simulink model "L2_scheme"  (R2026b)
settings: Solver=VariableStepAuto
settings Model: Creator=kiki  LastModifiedBy=kiki

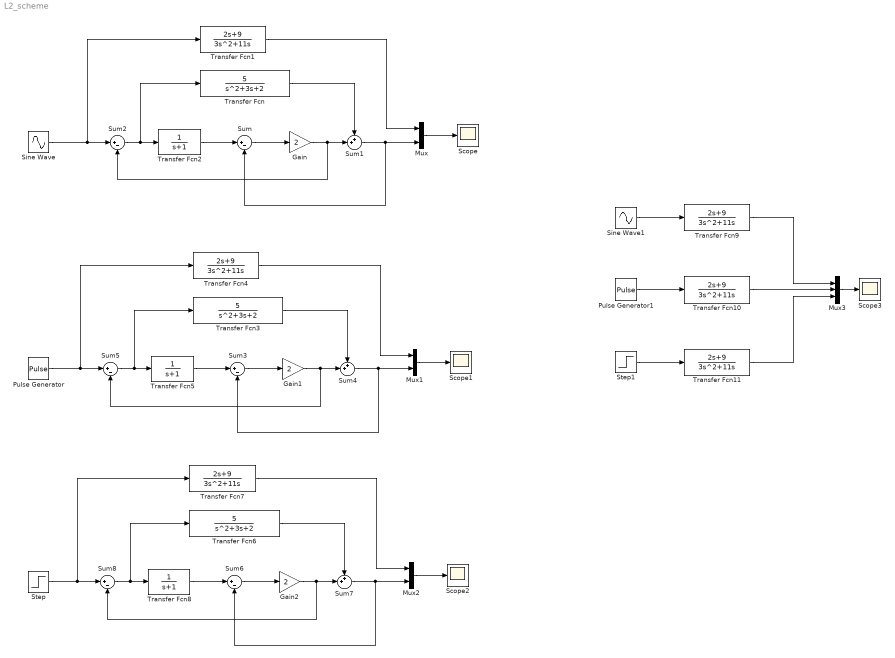
== system L2_scheme ==
  Gain : Gain  Gain=2
  Gain1 : Gain  Gain=2
  Gain2 : Gain  Gain=2
  Mux : Mux  Inputs=2
  Mux1 : Mux  Inputs=2
  Mux2 : Mux  Inputs=2
  Mux3 : Mux  Inputs=3
  Pulse Generator : DiscretePulseGenerator  PulseType=Time based  Period=10  PulseWidth=5
  Pulse Generator1 : DiscretePulseGenerator  PulseType=Time based  Period=10  PulseWidth=5
  Scope{,1..3} (4 alike) : Scope
      Scope settings: ActiveDisplayYMinimum=-0.20329483184246319  ActiveDisplayYMaximum=1.8296534865821692
      Scope1 settings: ActiveDisplayYMinimum=-0.20334831887683819  ActiveDisplayYMaximum=1.8301348698915443
      Scope2 settings: ActiveDisplayYMinimum=-0.20334831887683819  ActiveDisplayYMaximum=1.8301348698915443  DataLoggingVariableName=ScopeData2
      Scope3 settings: ActiveDisplayYMinimum=-0.91528925619834733  ActiveDisplayYMaximum=8.2376033057851288  DataLoggingVariableName=ScopeData3
  Sine Wave : Sin  SampleTime=0
  Sine Wave1 : Sin  SampleTime=0
  Step : Step  SampleTime=0
  Step1 : Step  SampleTime=0
  Sum{,2..3,5..6,8} (6 alike) : Sum  Inputs=|+-
  Sum1 : Sum  Inputs=++|
  Sum4 : Sum  Inputs=++|
  Sum7 : Sum  Inputs=++|
  Transfer Fcn : TransferFcn  Numerator=[5]  Denominator=[1 3 2]
  Transfer Fcn{1,4,7,9..11} (6 alike) : TransferFcn  Numerator=[2 9]  Denominator=[3 11 0]
  Transfer Fcn2 : TransferFcn  Denominator=[1 1]
  Transfer Fcn3 : TransferFcn  Numerator=[5]  Denominator=[1 3 2]
  Transfer Fcn5 : TransferFcn  Denominator=[1 1]
  Transfer Fcn6 : TransferFcn  Numerator=[5]  Denominator=[1 3 2]
  Transfer Fcn8 : TransferFcn  Denominator=[1 1]
  wires:
  Sum2/1 -> Transfer Fcn/1, Transfer Fcn2/1
  Transfer Fcn/1 -> Sum1/1
  Sum/1 -> Gain/1
  Transfer Fcn2/1 -> Sum/1
  Sum1/1 -> Mux/2, Sum/2
  Gain/1 -> Sum2/2, Sum1/2
  Sine Wave/1 -> Transfer Fcn1/1, Sum2/1
  Mux/1 -> Scope/1
  Transfer Fcn1/1 -> Mux/1
  Mux1/1 -> Scope1/1
  Sum3/1 -> Gain1/1
  Transfer Fcn4/1 -> Mux1/1
  Gain1/1 -> Sum5/2, Sum4/2
  Transfer Fcn5/1 -> Sum3/1
  Pulse Generator/1 -> Transfer Fcn4/1, Sum5/1
  Sum4/1 -> Mux1/2, Sum3/2
  Transfer Fcn3/1 -> Sum4/1
  Sum5/1 -> Transfer Fcn3/1, Transfer Fcn5/1
  Mux2/1 -> Scope2/1
  Sum6/1 -> Gain2/1
  Transfer Fcn7/1 -> Mux2/1
  Gain2/1 -> Sum8/2, Sum7/2
  Transfer Fcn8/1 -> Sum6/1
  Step/1 -> Transfer Fcn7/1, Sum8/1
  Sum7/1 -> Mux2/2, Sum6/2
  Transfer Fcn6/1 -> Sum7/1
  Sum8/1 -> Transfer Fcn6/1, Transfer Fcn8/1
  Step1/1 -> Transfer Fcn11/1
  Pulse Generator1/1 -> Transfer Fcn10/1
  Sine Wave1/1 -> Transfer Fcn9/1
  Transfer Fcn10/1 -> Mux3/2
  Transfer Fcn9/1 -> Mux3/1
  Transfer Fcn11/1 -> Mux3/3
  Mux3/1 -> Scope3/1
